simulink model "EMG_Prosthetic"  (R2026a)
settings: Solver=ode23tb  StopTime=P.Tstop  MaxStep=P.maxStep
values from neighbouring files (symbols this model uses):
  P = emg_params();  assignin('base','P',P)    [build_EMG_model.m]    (also in validate_EMG_model.m = emg_params())
settings Model: Creator=adity  LastModifiedBy=adity
settings DataIOCC: SaveFormat=StructureWithTime

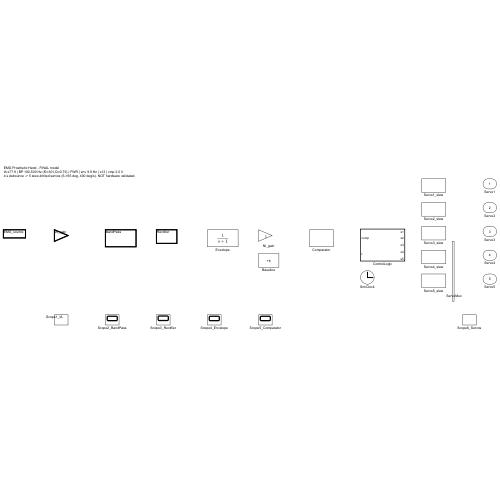
[thumbnail: Simulink's stored preview of the top-level diagram]
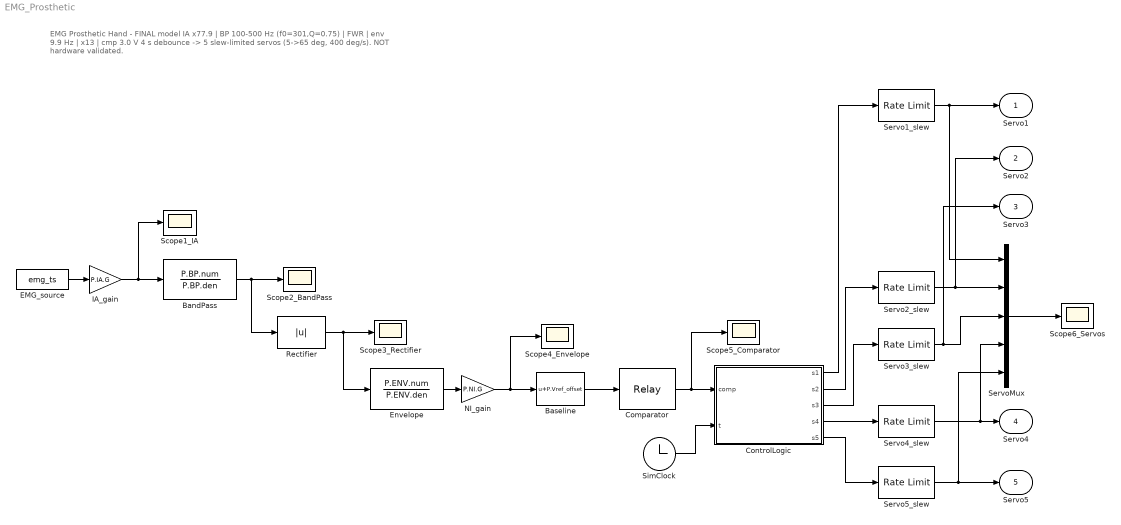
== system EMG_Prosthetic ==
  note: EMG Prosthetic Hand - FINAL model
      | IA x77.9 | BP 100-500 Hz (f0=301,Q=0.75) | FWR | env 9.9 Hz | x13 | cmp 3.0 V
      | 4 s debounce -> 5 slew-limited servos (5->65 deg, 400 deg/s). NOT hardware validated.
  BandPass : TransferFcn  Numerator=P.BP.num  Denominator=P.BP.den
  Baseline : Bias  Bias=P.Vref_offset  SaturateOnIntegerOverflow=off
  Comparator : Relay  OnSwitchValue=P.CMP.Vth + P.CMP.hyst  OffSwitchValue=P.CMP.Vth - P.CMP.hyst  OnOutputValue=P.CMP.Vhi  OffOutputValue=P.CMP.Vlo
  ControlLogic : MATLAB Function  TreatAsAtomicUnit=on
  EMG_source : FromWorkspace  VariableName=emg_ts
  Envelope : TransferFcn  Numerator=P.ENV.num  Denominator=P.ENV.den
  IA_gain : Gain  Gain=P.IA.G
  NI_gain : Gain  Gain=P.NI.G
  Rectifier : Abs  SaturateOnIntegerOverflow=off
  Scope1_IA : Scope
  Scope2_BandPass : Scope
  Scope3_Rectifier : Scope
  Scope4_Envelope : Scope
  Scope5_Comparator : Scope
  Scope6_Servos : Scope
  Servo1_slew : RateLimiter  RisingSlewLimit=P.SERVO.slew_dps  FallingSlewLimit=-P.SERVO.slew_dps  SampleTimeMode=inherited
  Servo2_slew : RateLimiter  RisingSlewLimit=P.SERVO.slew_dps  FallingSlewLimit=-P.SERVO.slew_dps  SampleTimeMode=inherited
  Servo3_slew : RateLimiter  RisingSlewLimit=P.SERVO.slew_dps  FallingSlewLimit=-P.SERVO.slew_dps  SampleTimeMode=inherited
  Servo4_slew : RateLimiter  RisingSlewLimit=P.SERVO.slew_dps  FallingSlewLimit=-P.SERVO.slew_dps  SampleTimeMode=inherited
  Servo5_slew : RateLimiter  RisingSlewLimit=P.SERVO.slew_dps  FallingSlewLimit=-P.SERVO.slew_dps  SampleTimeMode=inherited
  ServoMux : Mux  Inputs=5
  SimClock : Clock
  Servo1 : Outport
  Servo2 : Outport  Port=2
  Servo3 : Outport  Port=3
  Servo4 : Outport  Port=4
  Servo5 : Outport  Port=5
  wires:
  EMG_source/1 -> IA_gain/1
  IA_gain/1 -> Scope1_IA/1, BandPass/1
  BandPass/1 -> Rectifier/1, Scope2_BandPass/1
  Rectifier/1 -> Envelope/1, Scope3_Rectifier/1
  Baseline/1 -> Comparator/1
  NI_gain/1 -> Scope4_Envelope/1, Baseline/1
  Envelope/1 -> NI_gain/1
  SimClock/1 -> ControlLogic/2(t)
  Comparator/1 -> Scope5_Comparator/1, ControlLogic/1(comp)
  ControlLogic/1(s1) -> Servo1_slew/1
  ControlLogic/2(s2) -> Servo2_slew/1
  ControlLogic/3(s3) -> Servo3_slew/1
  ControlLogic/4(s4) -> Servo4_slew/1
  Servo1_slew/1 -> ServoMux/1, Servo1/1
  ControlLogic/5(s5) -> Servo5_slew/1
  Servo2_slew/1 -> Servo2/1, ServoMux/2
  Servo3_slew/1 -> Servo3/1, ServoMux/3
  Servo4_slew/1 -> Servo4/1, ServoMux/4
  Servo5_slew/1 -> Servo5/1, ServoMux/5
  ServoMux/1 -> Scope6_Servos/1

== matlab function EMG_Prosthetic/ControlLogic ==
  data: comp input; s1 output; t input; s2 output; s3 output; s4 output; s5 output
function [s1,s2,s3,s4,s5] = ControlLogic(comp, t)
%#codegen
% One accepted contraction toggles the hand; a 4 s buffer rejects the
% multiple HIGH pulses of one contraction. Outputs five commanded servo
% angles (coordinated). Per-finger closed angles allow a natural grip.
persistent motorOn last
if isempty(motorOn), motorOn = false; last = -1e9; end
openA   = 5;                        %% servo.write(5)
closeV  = [65 65 65 65 65];         %% per-finger closed angles
deb     = 4;                        %% debounceDuration = 4000 ms
if comp > 2.5 && (t - last) > deb
    last = t;  motorOn = ~motorOn;
end
if motorOn, a = closeV; else, a = [openA openA openA openA openA]; end
s1 = a(1); s2 = a(2); s3 = a(3); s4 = a(4); s5 = a(5);
end
